simulink model "SR_Bench"  (R2024b)
settings: Solver=ode4  StartTime=0.0  StopTime=BP.Tend  FixedStep=BP.Ts  RelTol=1e-3
InitFcn:
  | sr_params_bench;
undefined symbols (not defined in the file): BP, BX
settings Model: Creator=sange  LastModifiedBy=sange
settings DataIOCC: SaveOutput=off

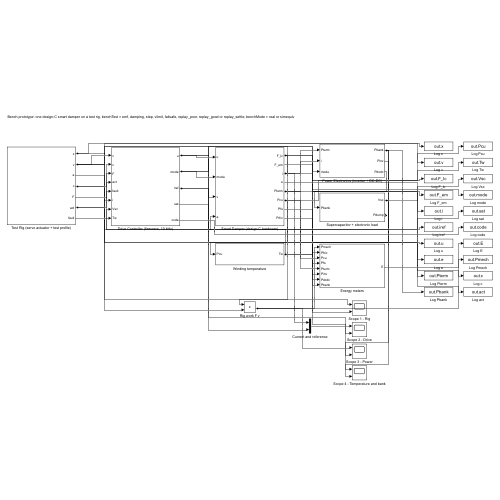
[thumbnail: Simulink's stored preview of the top-level diagram]
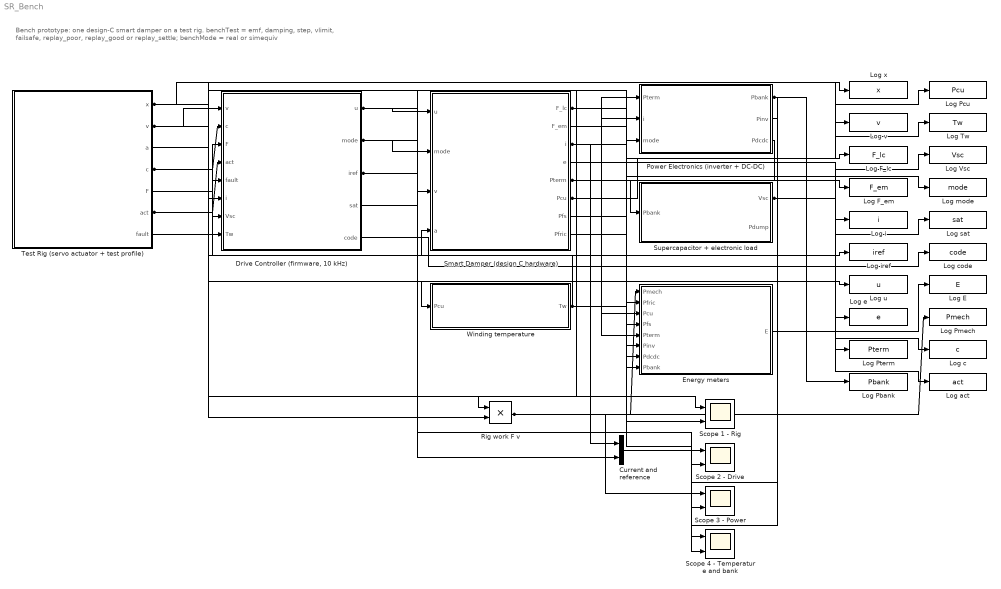
== system SR_Bench ==
  note: Bench prototype: one design-C smart damper on a test rig. benchTest = emf, damping, step, vlimit, failsafe, replay_poor, replay_good or replay_settle; benchMode = real or simequiv
  Current and reference : Mux  Inputs=2
  "Drive Controller (firmware, 10 kHz)" : Subsystem  Description=What the drive's microcontroller does every 100 us: fail-safe supervisor, current reference (damping law or push), PI current control with back-EMF feed-forward and voltage limit. Same algorithms as the C firmware (functions/bp_*.m = firmware/src/*.c).
  Energy meters : Subsystem  Description=Integrates every power flow so the energy balance can be checked: rig work in = friction + copper + fail-safe resistors + inverter + DC-DC + bank + stored (rotor, coil).
  Log E : ToWorkspace  VariableName=E  SaveFormat=Timeseries  SampleTime=BP.Tlog
  Log F_em : ToWorkspace  VariableName=F_em  SaveFormat=Timeseries  SampleTime=BP.Tlog
  Log F_lc : ToWorkspace  VariableName=F_lc  SaveFormat=Timeseries  SampleTime=BP.Tlog
  Log Pbank : ToWorkspace  VariableName=Pbank  SaveFormat=Timeseries  SampleTime=BP.Tlog
  Log Pcu : ToWorkspace  VariableName=Pcu  SaveFormat=Timeseries  SampleTime=BP.Tlog
  Log Pmech : ToWorkspace  VariableName=Pmech  SaveFormat=Timeseries  SampleTime=BP.Tlog
  Log Pterm : ToWorkspace  VariableName=Pterm  SaveFormat=Timeseries  SampleTime=BP.Tlog
  Log Tw : ToWorkspace  VariableName=Tw  SaveFormat=Timeseries  SampleTime=BP.Tlog
  Log Vsc : ToWorkspace  VariableName=Vsc  SaveFormat=Timeseries  SampleTime=BP.Tlog
  Log act : ToWorkspace  VariableName=act  SaveFormat=Timeseries  SampleTime=BP.Tlog
  Log c : ToWorkspace  VariableName=c  SaveFormat=Timeseries  SampleTime=BP.Tlog
  Log code : ToWorkspace  VariableName=code  SaveFormat=Timeseries  SampleTime=BP.Tlog
  Log e : ToWorkspace  VariableName=e  SaveFormat=Timeseries  SampleTime=BP.Tlog
  Log i : ToWorkspace  VariableName=i  SaveFormat=Timeseries  SampleTime=BP.Tlog
  Log iref : ToWorkspace  VariableName=iref  SaveFormat=Timeseries  SampleTime=BP.Tlog
  Log mode : ToWorkspace  VariableName=mode  SaveFormat=Timeseries  SampleTime=BP.Tlog
  Log sat : ToWorkspace  VariableName=sat  SaveFormat=Timeseries  SampleTime=BP.Tlog
  Log u : ToWorkspace  VariableName=u  SaveFormat=Timeseries  SampleTime=BP.Tlog
  Log v : ToWorkspace  VariableName=v  SaveFormat=Timeseries  SampleTime=BP.Tlog
  Log x : ToWorkspace  VariableName=x  SaveFormat=Timeseries  SampleTime=BP.Tlog
  Power Electronics (inverter + DC-DC) : Subsystem  Description=3-phase inverter (conduction and switching losses) and the bidirectional DC-DC converter that holds the 60 V DC link and charges the supercapacitor (12-48 V).
  Rig work F v : Product
  Scope 1 - Rig : Scope  NumInputPorts=2
  Scope 2 - Drive : Scope  NumInputPorts=2
  Scope 3 - Power : Scope  NumInputPorts=2
  Scope 4 - Temperature and bank : Scope  NumInputPorts=2
  Smart Damper (design C hardware) : Subsystem  Description=Design-C damper: ball screw turns the 3-phase servo machine (modelled as its equivalent DC machine: e = Ke v, F = Ke i, L di/dt = e - Rc i - u). The changeover contactor connects the coil to the inverter (normal) or to the fail-safe resistors (dropped). Friction and rotor inertance add to the force.
  Supercapacitor + electronic load : Subsystem  Description=The bogie's 10 F supercapacitor (one damper charges it on the bench) and an electronic load drawing this damper's half of the 8 W bogie electronics.
  Test Rig (servo actuator + test profile) : Subsystem  Description=Displacement-controlled actuator that strokes the damper (x, v, a) and the test computer that sends the drive its commands: damping c, push force F, push window act, test fault.
  Winding temperature : Subsystem  Description=First-order thermal model of the motor winding: copper loss in, heat out to ambient.
  wires:
  Test Rig (servo actuator + test profile)/2(v) -> "Drive Controller (firmware, 10 kHz)"/1(v), Smart Damper (design C hardware)/3(v), Rig work F v/2, Log v/1
  Test Rig (servo actuator + test profile)/4(c) -> "Drive Controller (firmware, 10 kHz)"/2(c), Log c/1
  Test Rig (servo actuator + test profile)/5(F) -> "Drive Controller (firmware, 10 kHz)"/3(F)
  Test Rig (servo actuator + test profile)/6(act) -> "Drive Controller (firmware, 10 kHz)"/4(act), Log act/1
  Test Rig (servo actuator + test profile)/7(fault) -> "Drive Controller (firmware, 10 kHz)"/5(fault)
  Smart Damper (design C hardware)/3(i) -> "Drive Controller (firmware, 10 kHz)"/6(i), Power Electronics (inverter + DC-DC)/2(i), Log i/1, Current and reference/1
  Supercapacitor + electronic load/1(Vsc) -> "Drive Controller (firmware, 10 kHz)"/7(Vsc), Log Vsc/1, Scope 4 - Temperature and bank/2
  Winding temperature/1(Tw) -> "Drive Controller (firmware, 10 kHz)"/8(Tw), Log Tw/1, Scope 4 - Temperature and bank/1
  "Drive Controller (firmware, 10 kHz)"/1(u) -> Smart Damper (design C hardware)/1(u), Log u/1, Scope 2 - Drive/2
  "Drive Controller (firmware, 10 kHz)"/2(mode) -> Smart Damper (design C hardware)/2(mode), Power Electronics (inverter + DC-DC)/3(mode), Log mode/1
  Test Rig (servo actuator + test profile)/3(a) -> Smart Damper (design C hardware)/4(a)
  Smart Damper (design C hardware)/5(Pterm) -> Power Electronics (inverter + DC-DC)/1(Pterm), Energy meters/5(Pterm), Log Pterm/1
  Power Electronics (inverter + DC-DC)/1(Pbank) -> Supercapacitor + electronic load/1(Pbank), Energy meters/8(Pbank), Log Pbank/1, Scope 3 - Power/2
  Smart Damper (design C hardware)/6(Pcu) -> Winding temperature/1(Pcu), Energy meters/3(Pcu), Log Pcu/1
  Smart Damper (design C hardware)/1(F_lc) -> Rig work F v/1, Log F_lc/1, Scope 1 - Rig/2
  Rig work F v/1 -> Energy meters/1(Pmech), Log Pmech/1, Scope 3 - Power/1
  Smart Damper (design C hardware)/8(Pfric) -> Energy meters/2(Pfric)
  Smart Damper (design C hardware)/7(Pfs) -> Energy meters/4(Pfs)
  Power Electronics (inverter + DC-DC)/2(Pinv) -> Energy meters/6(Pinv)
  Power Electronics (inverter + DC-DC)/3(Pdcdc) -> Energy meters/7(Pdcdc)
  Test Rig (servo actuator + test profile)/1(x) -> Log x/1, Scope 1 - Rig/1
  Smart Damper (design C hardware)/2(F_em) -> Log F_em/1
  "Drive Controller (firmware, 10 kHz)"/3(iref) -> Log iref/1, Current and reference/2
  Smart Damper (design C hardware)/4(e) -> Log e/1
  "Drive Controller (firmware, 10 kHz)"/4(sat) -> Log sat/1
  "Drive Controller (firmware, 10 kHz)"/5(code) -> Log code/1
  Energy meters/1(E) -> Log E/1
  Current and reference/1 -> Scope 2 - Drive/1

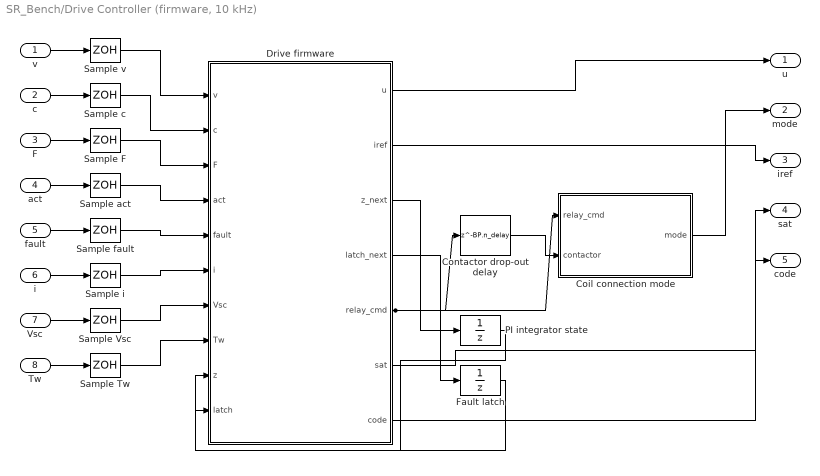
== system SR_Bench/Drive Controller (firmware, 10 kHz) ==
  v : Inport
  c : Inport  Port=2
  F : Inport  Port=3
  act : Inport  Port=4
  fault : Inport  Port=5
  i : Inport  Port=6
  Vsc : Inport  Port=7
  Tw : Inport  Port=8
  Coil connection mode : MATLAB Function  TreatAsAtomicUnit=on
  Contactor drop-out delay : Delay  DelayLength=BP.n_delay  InitialCondition=0  SampleTime=BP.Ti
  Drive firmware : MATLAB Function  TreatAsAtomicUnit=on
  Fault latch : UnitDelay  SampleTime=BP.Ti  HasFrameUpgradeWarning=on
  PI integrator state : UnitDelay  SampleTime=BP.Ti  HasFrameUpgradeWarning=on
  Sample F : ZeroOrderHold  SampleTime=BP.Ti
  Sample Tw : ZeroOrderHold  SampleTime=BP.Ti
  Sample Vsc : ZeroOrderHold  SampleTime=BP.Ti
  Sample act : ZeroOrderHold  SampleTime=BP.Ti
  Sample c : ZeroOrderHold  SampleTime=BP.Ti
  Sample fault : ZeroOrderHold  SampleTime=BP.Ti
  Sample i : ZeroOrderHold  SampleTime=BP.Ti
  Sample v : ZeroOrderHold  SampleTime=BP.Ti
  u : Outport
  mode : Outport  Port=2
  iref : Outport  Port=3
  sat : Outport  Port=4
  code : Outport  Port=5
  wires:
  v/1 -> Sample v/1
  c/1 -> Sample c/1
  F/1 -> Sample F/1
  act/1 -> Sample act/1
  fault/1 -> Sample fault/1
  i/1 -> Sample i/1
  Vsc/1 -> Sample Vsc/1
  Tw/1 -> Sample Tw/1
  Sample v/1 -> Drive firmware/1(v)
  Sample c/1 -> Drive firmware/2(c)
  Sample F/1 -> Drive firmware/3(F)
  Sample act/1 -> Drive firmware/4(act)
  Sample fault/1 -> Drive firmware/5(fault)
  Sample i/1 -> Drive firmware/6(i)
  Sample Vsc/1 -> Drive firmware/7(Vsc)
  Sample Tw/1 -> Drive firmware/8(Tw)
  PI integrator state/1 -> Drive firmware/9(z)
  Fault latch/1 -> Drive firmware/10(latch)
  Drive firmware/3(z_next) -> PI integrator state/1
  Drive firmware/4(latch_next) -> Fault latch/1
  Drive firmware/5(relay_cmd) -> Contactor drop-out delay/1, Coil connection mode/1(relay_cmd)
  Contactor drop-out delay/1 -> Coil connection mode/2(contactor)
  Drive firmware/1(u) -> u/1
  Coil connection mode/1(mode) -> mode/1
  Drive firmware/2(iref) -> iref/1
  Drive firmware/6(sat) -> sat/1
  Drive firmware/7(code) -> code/1

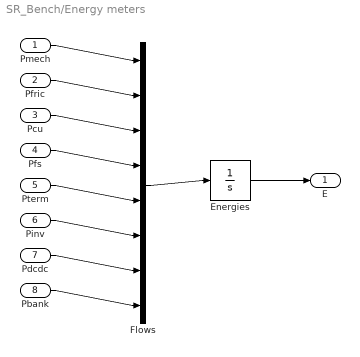
== system SR_Bench/Energy meters ==
  Pmech : Inport
  Pfric : Inport  Port=2
  Pcu : Inport  Port=3
  Pfs : Inport  Port=4
  Pterm : Inport  Port=5
  Pinv : Inport  Port=6
  Pdcdc : Inport  Port=7
  Pbank : Inport  Port=8
  Energies : Integrator  InitialCondition=zeros(8,1)
  Flows : Mux  Inputs=8
  E : Outport
  wires:
  Pmech/1 -> Flows/1
  Pfric/1 -> Flows/2
  Pcu/1 -> Flows/3
  Pfs/1 -> Flows/4
  Pterm/1 -> Flows/5
  Pinv/1 -> Flows/6
  Pdcdc/1 -> Flows/7
  Pbank/1 -> Flows/8
  Flows/1 -> Energies/1
  Energies/1 -> E/1

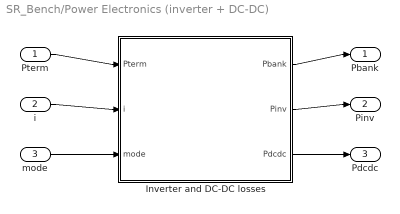
== system SR_Bench/Power Electronics (inverter + DC-DC) ==
  Pterm : Inport
  i : Inport  Port=2
  mode : Inport  Port=3
  Inverter and DC-DC losses : MATLAB Function  TreatAsAtomicUnit=on
  Pbank : Outport
  Pinv : Outport  Port=2
  Pdcdc : Outport  Port=3
  wires:
  Inverter and DC-DC losses/1(Pbank) -> Pbank/1
  Inverter and DC-DC losses/2(Pinv) -> Pinv/1
  Inverter and DC-DC losses/3(Pdcdc) -> Pdcdc/1
  Pterm/1 -> Inverter and DC-DC losses/1(Pterm)
  i/1 -> Inverter and DC-DC losses/2(i)
  mode/1 -> Inverter and DC-DC losses/3(mode)

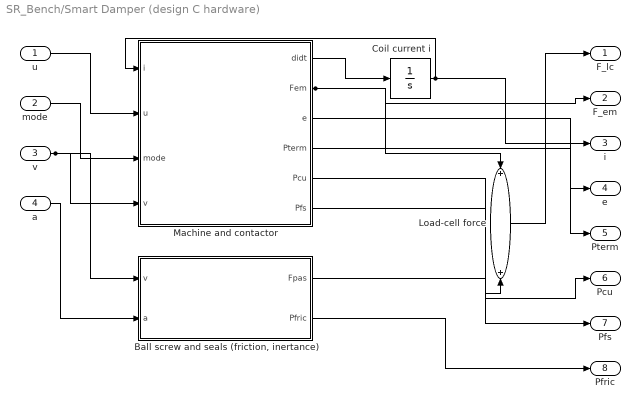
== system SR_Bench/Smart Damper (design C hardware) ==
  u : Inport
  mode : Inport  Port=2
  v : Inport  Port=3
  a : Inport  Port=4
  "Ball screw and seals (friction, inertance)" : MATLAB Function  TreatAsAtomicUnit=on
  Coil current i : Integrator
  Load-cell force : Sum
  Machine and contactor : MATLAB Function  TreatAsAtomicUnit=on
  F_lc : Outport
  F_em : Outport  Port=2
  i : Outport  Port=3
  e : Outport  Port=4
  Pterm : Outport  Port=5
  Pcu : Outport  Port=6
  Pfs : Outport  Port=7
  Pfric : Outport  Port=8
  wires:
  Coil current i/1 -> Machine and contactor/1(i), i/1
  u/1 -> Machine and contactor/2(u)
  mode/1 -> Machine and contactor/3(mode)
  v/1 -> Machine and contactor/4(v), "Ball screw and seals (friction, inertance)"/1(v)
  Machine and contactor/1(didt) -> Coil current i/1
  a/1 -> "Ball screw and seals (friction, inertance)"/2(a)
  Machine and contactor/2(Fem) -> Load-cell force/1, F_em/1
  "Ball screw and seals (friction, inertance)"/1(Fpas) -> Load-cell force/2
  Load-cell force/1 -> F_lc/1
  Machine and contactor/3(e) -> e/1
  Machine and contactor/4(Pterm) -> Pterm/1
  Machine and contactor/5(Pcu) -> Pcu/1
  Machine and contactor/6(Pfs) -> Pfs/1
  "Ball screw and seals (friction, inertance)"/2(Pfric) -> Pfric/1

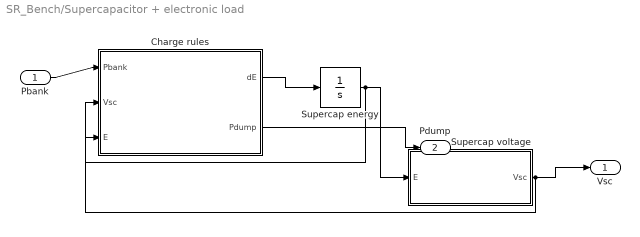
== system SR_Bench/Supercapacitor + electronic load ==
  Pbank : Inport
  Charge rules : MATLAB Function  TreatAsAtomicUnit=on
  Supercap energy : Integrator  InitialCondition=BP.Esc0
  Supercap voltage : MATLAB Function  TreatAsAtomicUnit=on
  Vsc : Outport
  Pdump : Outport  Port=2
  wires:
  Pbank/1 -> Charge rules/1(Pbank)
  Supercap energy/1 -> Supercap voltage/1(E), Charge rules/3(E)
  Supercap voltage/1(Vsc) -> Charge rules/2(Vsc), Vsc/1
  Charge rules/1(dE) -> Supercap energy/1
  Charge rules/2(Pdump) -> Pdump/1

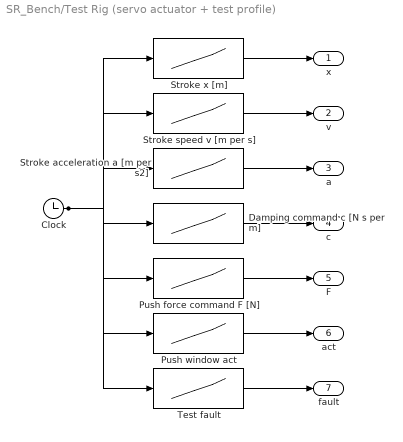
== system SR_Bench/Test Rig (servo actuator + test profile) ==
  Clock : Clock
  Damping command c [N s per m] : Lookup_n-D  NumberOfTableDimensions=1  BreakpointsForDimension1=BX.t  Table=BX.c  ExtrapMethod=Clip  InternalRulePriority=Speed  RndMeth=Simplest
  Push force command F [N] : Lookup_n-D  NumberOfTableDimensions=1  BreakpointsForDimension1=BX.t  Table=BX.F  ExtrapMethod=Clip  InternalRulePriority=Speed  RndMeth=Simplest
  Push window act : Lookup_n-D  NumberOfTableDimensions=1  BreakpointsForDimension1=BX.t  Table=BX.act  InterpMethod=Flat  ExtrapMethod=Clip  InternalRulePriority=Speed  RndMeth=Simplest
  Stroke acceleration a [m per s2] : Lookup_n-D  NumberOfTableDimensions=1  BreakpointsForDimension1=BX.t  Table=BX.a  ExtrapMethod=Clip  InternalRulePriority=Speed  RndMeth=Simplest
  Stroke speed v [m per s] : Lookup_n-D  NumberOfTableDimensions=1  BreakpointsForDimension1=BX.t  Table=BX.v  ExtrapMethod=Clip  InternalRulePriority=Speed  RndMeth=Simplest
  Stroke x [m] : Lookup_n-D  NumberOfTableDimensions=1  BreakpointsForDimension1=BX.t  Table=BX.x  ExtrapMethod=Clip  InternalRulePriority=Speed  RndMeth=Simplest
  Test fault : Lookup_n-D  NumberOfTableDimensions=1  BreakpointsForDimension1=BX.t  Table=BX.fault  InterpMethod=Flat  ExtrapMethod=Clip  InternalRulePriority=Speed  RndMeth=Simplest
  x : Outport
  v : Outport  Port=2
  a : Outport  Port=3
  c : Outport  Port=4
  F : Outport  Port=5
  act : Outport  Port=6
  fault : Outport  Port=7
  wires:
  Clock/1 -> Stroke x [m]/1, Stroke speed v [m per s]/1, Stroke acceleration a [m per s2]/1, Damping command c [N s per m]/1, Push force command F [N]/1, Push window act/1, Test fault/1
  Stroke x [m]/1 -> x/1
  Stroke speed v [m per s]/1 -> v/1
  Stroke acceleration a [m per s2]/1 -> a/1
  Damping command c [N s per m]/1 -> c/1
  Push force command F [N]/1 -> F/1
  Push window act/1 -> act/1
  Test fault/1 -> fault/1

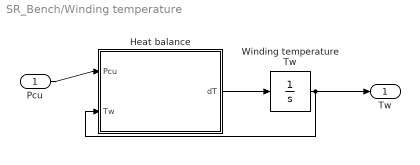
== system SR_Bench/Winding temperature ==
  Pcu : Inport
  Heat balance : MATLAB Function  TreatAsAtomicUnit=on
  Winding temperature Tw : Integrator  InitialCondition=BP.Tw0
  Tw : Outport
  wires:
  Pcu/1 -> Heat balance/1(Pcu)
  Winding temperature Tw/1 -> Heat balance/2(Tw), Tw/1
  Heat balance/1(dT) -> Winding temperature Tw/1

== matlab function SR_Bench/Supercapacitor + electronic load/Charge rules ==
  data: Pbank input; dE output; Vsc input; E input; Pdump output; BP parameter
function [dE, Pdump] = fcn(Pbank, Vsc, E, BP)
p = Pbank - BP.Pload;
Pdump = 0;
if Vsc >= BP.Vmax && p > 0
    Pdump = p;  p = 0;                               % full: the surplus goes to a dump resistor
end
if E <= 0 && p < 0
    p = 0;
end
dE = p;

== matlab function SR_Bench/Winding temperature/Heat balance ==
  data: Pcu input; dT output; Tw input; BP parameter
function dT = fcn(Pcu, Tw, BP)
dT = (Pcu - (Tw - BP.Tamb) / BP.Rth) / BP.Cth;

== matlab function SR_Bench/Drive Controller (firmware, 10 kHz)/Coil connection mode ==
  data: relay_cmd input; mode output; contactor input
function mode = fcn(relay_cmd, contactor)
% 0 = inverter drives the coil.  1 = gates off, contactor still moving (coil open).
% 2 = contactor dropped: coil on the fail-safe resistors (today's passive damping).
if contactor > 0.5
    mode = 2;
elseif relay_cmd > 0.5
    mode = 1;
else
    mode = 0;
end

== matlab function SR_Bench/Drive Controller (firmware, 10 kHz)/Drive firmware ==
  data: v input; u output; c input; F input; act input; fault input; i input; Vsc input; Tw input; z input; latch input; iref output; z_next output; latch_next output; relay_cmd output; sat output; code output; BP parameter
function [u, iref, z_next, latch_next, relay_cmd, sat, code] = fcn(v, c, F, act, fault, i, Vsc, Tw, z, latch, BP)
% 1. Fail-safe supervisor (drops the contactor on a fault, latched).
% 2. Current reference: damping law i = c v / Ke, or the push force inside a window.
% 3. PI current control + back-EMF feed-forward, limited to the inverter voltage.
[relay_cmd, latch_next, code] = bp_failsafe(fault, Vsc, Tw, i, latch, BP);
iref = bp_current_ref(c, F, act, v, BP);
[u, z_next, sat] = bp_current_ctrl(iref, i, v, z, BP);
if relay_cmd > 0.5
    u = 0;  z_next = 0;  iref = 0;  sat = 0;    % gates off: the contactor takes over
end

== matlab function SR_Bench/Smart Damper (design C hardware)/Machine and contactor ==
  data: i input; u input; didt output; mode input; v input; Fem output; e output; Pterm output; Pcu output; Pfs output; BP parameter
function [didt, Fem, e, Pterm, Pcu, Pfs] = fcn(i, u, mode, v, BP)
% Equivalent DC machine. Pterm: power delivered to the inverter terminals.
e = BP.Ke * v;
if mode > 1.5
    didt = (e - (BP.Rc + BP.R_fs) * i) / BP.L;      % coil on the fail-safe resistors
    Pterm = 0;  Pfs = BP.R_fs * i^2;
elseif mode > 0.5
    didt = -i / BP.tau_open;                          % gates off: current collapses through the diodes
    Pterm = (e - BP.Rc * i - BP.L * didt) * i;  Pfs = 0;
else
    didt = (e - BP.Rc * i - u) / BP.L;                % inverter applies u
    Pterm = u * i;  Pfs = 0;
end
Fem = BP.Ke * i;
Pcu = BP.Rc * i^2;

== matlab function SR_Bench/Smart Damper (design C hardware)/Ball screw and seals (friction, inertance) ==
  data: v input; Fpas output; a input; Pfric output; BP parameter
function [Fpas, Pfric] = fcn(v, a, BP)
Ffr = BP.Fc * tanh(v / BP.veps);                     % screw + seal friction
Fpas = Ffr + BP.b_in * a;                            % rotor + screw inertia seen at the rod
Pfric = Ffr * v;

== matlab function SR_Bench/Power Electronics (inverter + DC-DC)/Inverter and DC-DC losses ==
  data: Pterm input; Pbank output; i input; mode input; Pinv output; Pdcdc output; BP parameter
function [Pbank, Pinv, Pdcdc] = fcn(Pterm, i, mode, BP)
Pinv = 0;
if mode < 0.5
    Pinv = BP.Ron * i^2 + BP.ksw * abs(i);            % conduction + switching
end
Plink = Pterm - Pinv;
Pbank = BP.eta_dcdc * max(Plink, 0) + min(Plink, 0) / BP.eta_dcdc;
Pdcdc = Plink - Pbank;

== matlab function SR_Bench/Supercapacitor + electronic load/Supercap voltage ==
  data: E input; Vsc output; BP parameter
function Vsc = fcn(E, BP)
Vsc = sqrt(max(2 * E / BP.Csc, 0));
